simulink library "atmosphere_lib"  (R2018b)
settings: Solver=VariableStepAuto  StartTime=0.0  StopTime=10.0  RelTol=1e-3
values from neighbouring files (symbols this model uses):
  wg = interp1(y',wg_big',Y)'    [vonKarman2D.m]
  x = 0:Delta_x:x_max    [vonKarman1D.m]    (also in vonKarman2D.m)
undefined symbols (not defined in the file or in its folder): DiscIntNeverNeededParam
libraries: simulink x3, linear_systems_lib x3
settings Model: Creator=Ybeyer  LastModifiedBy=yannic
settings DebuggingCC: LibraryContextMissingDiagnostic=none
settings SFSimCC: SimUseLocalCustomCode=off
settings RTWCC: RTWUseLocalCustomCode=off
settings CodeAppCC: StateflowObjectComments=on

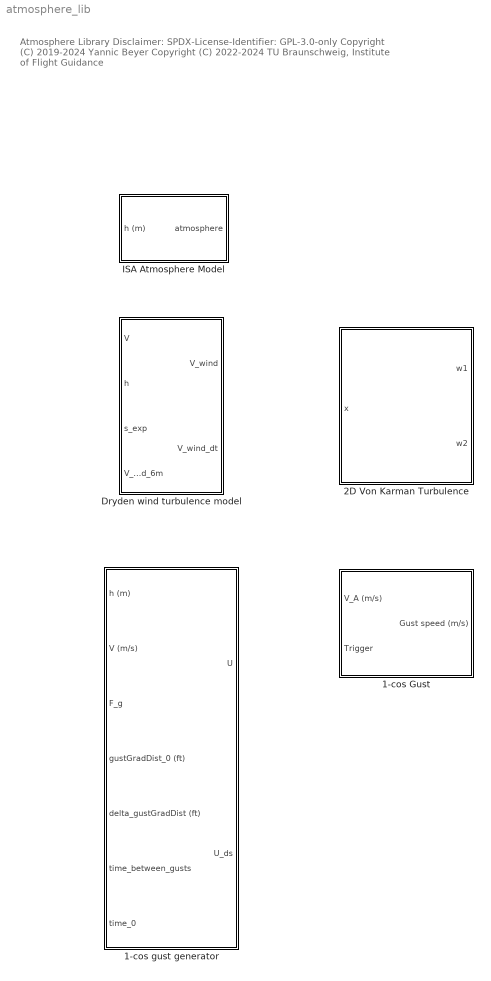
== system atmosphere_lib ==
  note: Atmosphere Library
      |
      | Disclaimer:
      | SPDX-License-Identifier: GPL-3.0-only
      |
      | Copyright (C) 2019-2024 Yannic Beyer
      | Copyright (C) 2022-2024 TU Braunschweig, Institute of Flight Guidance
  1-cos Gust : Subsystem  mask{gust_magnitude=3, gust_length=20}
      mask prompts: gust_magnitude "Gust magnitude, in m/s"; gust_length "Gust length, in m"
      mask DialogControl DescGroupVar Prompt: 1-cos gust
      mask DialogControl DescTextVar Prompt: This block creates 1-cos gust speeds.
  1-cos gust generator : Subsystem
      mask DialogControl DescGroupVar Prompt: 1-cos gust generator
      mask DialogControl DescTextVar Prompt: With this block you can generate a time series of 1-cos gusts. You can use the inputs to specify parameters like the initial gust gradient distance and how you want to increment the gust gradient distance for the next gust. Moreover, you can specify the time between the gusts.
      mask DialogControl ParameterGroupVar Prompt: Inputs
      mask DialogControl Control2 Prompt: h - altitude (m)
      mask DialogControl Control3 Prompt: V - airspeed of the aircraft (m/s)
      mask DialogControl Control4 Prompt: F_g - flight profile alleviation factor
      mask DialogControl Control5 Prompt: gustGradDist_0 - initial gust gradient distance (m)
      mask DialogControl Control6 Prompt: delta_gustGradDist - difference of the gust gradient distance for the next gust (m)
      mask DialogControl Control7 Prompt: time_between gusts - the time between gusts where there will be no wind (s)
      mask DialogControl Control8 Prompt: time_0 - time when the first gust starts
  2D Von Karman Turbulence : Subsystem  mask{x_max=10000, y_max=2*762, Delta_x=1, Delta_y=1, sigma=6.5, L=762, Y={[-2,-1,0,1,2],[-10,-5,0,5,10]}, is_symmetric=on, seed=2}
      mask prompts: x_max "Longitudinal length (m) - should be higher than scale length"; y_max "Lateral width (m) - should be higher than scale length"; Delta_x "Longitudinal position resolution (m)"; Delta_y "Lateral position resolution (m)"; sigma "Turbulence velocity variance (m/s), see turbulenceIntensityRMS"; L "Scale length at medium/high altitudes (m)"; Y "Lateral positions of interest (m)"; is_symmetric "Should the wind field be symmetric in lateral direction?"; seed "Noise seed"
      mask init:
      | y = [];
      | len = [];
      | for i = 1:length(Y)
      |     y(end+1:end+length(Y{i})) = Y{i};
      |     len(end+1) = length(Y{i});
      | end
      | [wg,wg_big,x] = vonKarman2D( x_max, y_max, Delta_x, Delta_y, y, sigma, L, seed, is_symmetric );
      | assignin('base','wind2D',wg);
      | assignin('base','wind2D_big',wg_big);
      | vonKarman2DInitBlock(gcb,len);
      mask DialogControl DescGroupVar Prompt: 2D von Kármán turbulence wind field
      mask DialogControl DescTextVar Prompt: For the 2D turbulence field no only computation via a white noise generator and a filter could be found. Instead, the wind field is computed during initialization with a 2D fourier transform according to literature.
      mask DialogControl Control2 Prompt: The whole wind field is saved to the base workspace as "wind2D_big". The wind field for the lateral positions of interest is saved as "wind2D".
  Dryden wind turbulence model : Subsystem  mask{noise_sample_time=0.01, noise_seed=[23341,23342,23343]}
      mask prompts: noise_sample_time "band-limited white noise sample time"; noise_seed "band-limited white noise seed"
      mask DialogControl DescTextVar Prompt: Inputs:
      mask DialogControl Control2 Prompt: V   - airspeed, m/s
      mask DialogControl Control3 Prompt: h   - altitude, m
      mask DialogControl Control4 Prompt: s_exp   - severity exponent (-1...6)
      mask DialogControl Control5 Prompt: V_wind   - wind velocity 6m above ground
  ISA Atmosphere Model : Subsystem
      mask init:
      | % init atmosphere struct
      | atmosphere = isAtmosphere(0);
      | % create bus object in base workspace
      | struct2bus(atmosphere);
      mask DialogControl DescGroupVar Prompt: International Standard Atmosphere Model
      mask DialogControl DescTextVar Prompt: The output is a bus (bus object is created in base workspace) and all quantities are in SI units.

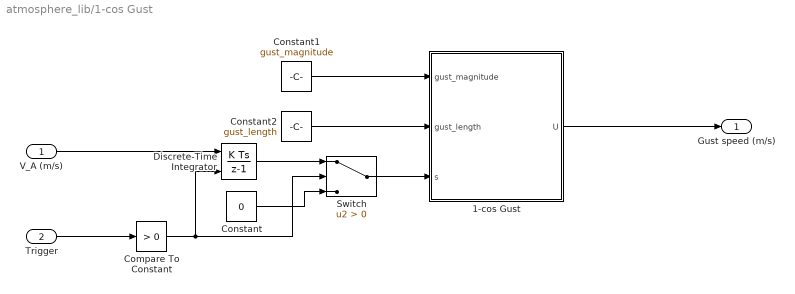
== system atmosphere_lib/1-cos Gust ==
  V_A (m/s) : Inport
  Trigger : Inport  Port=2
  1-cos Gust : MATLAB Function  TreatAsAtomicUnit=on
  Compare To Constant : simulink/Logic and Bit Operations/Compare To Constant  relop=>  const=0  OutDataTypeStr=boolean
  Constant : Constant  Value=0
  Constant1 : Constant  Value=gust_magnitude
  Constant2 : Constant  Value=gust_length
  Discrete-Time Integrator : DiscreteIntegrator  ExternalReset=rising  SampleTime=-1  ICPrevOutput=DiscIntNeverNeededParam  ICPrevScaledInput=DiscIntNeverNeededParam
  Switch : Switch  Criteria=u2 > Threshold
  Gust speed (m/s) : Outport
  wires:
  V_A (m/s)/1 -> Discrete-Time Integrator/1
  Constant2/1 -> 1-cos Gust/2(gust_length)
  Discrete-Time Integrator/1 -> Switch/1
  Trigger/1 -> Compare To Constant/1
  Compare To Constant/1 -> Switch/2, Discrete-Time Integrator/2
  Switch/1 -> 1-cos Gust/3(s)
  Constant/1 -> Switch/3
  1-cos Gust/1(U) -> Gust speed (m/s)/1
  Constant1/1 -> 1-cos Gust/1(gust_magnitude)

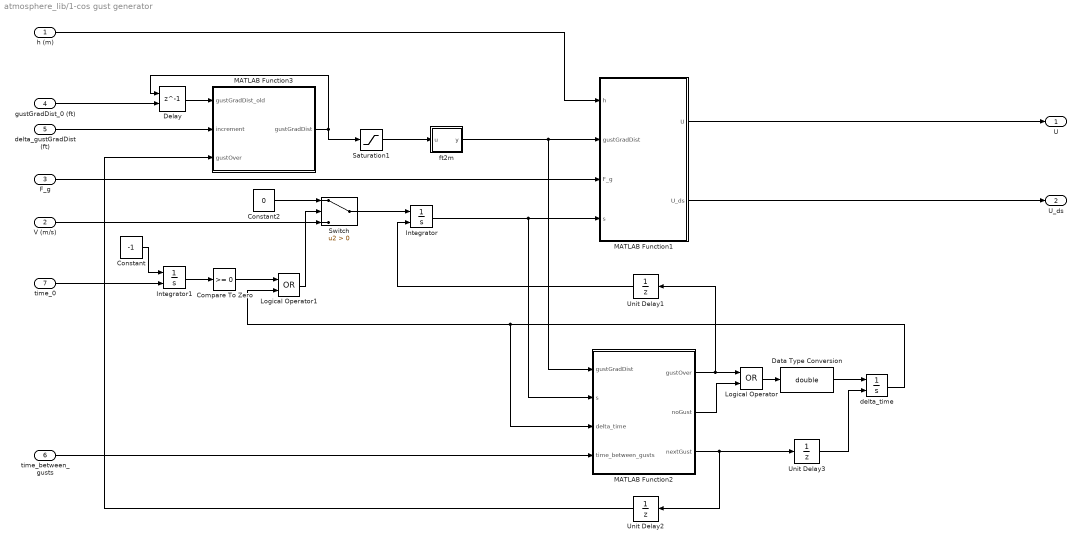
== system atmosphere_lib/1-cos gust generator ==
  h (m) : Inport
  V (m/s) : Inport  Port=2
  F_g : Inport  Port=3
  gustGradDist_0 (ft) : Inport  Port=4
  delta_gustGradDist (ft) : Inport  Port=5
  time_between_gusts : Inport  Port=6
  time_0 : Inport  Port=7
  Compare To Zero : simulink/Logic and Bit Operations/Compare To Zero  relop=>=  OutDataTypeStr=boolean
  Constant : Constant  Value=-1
  Constant2 : Constant  Value=0
  Data Type Conversion : DataTypeConversion  OutDataTypeStr=double
  Delay : Delay  DelayLength=1  InitialConditionSource=Input port
      settings: InputPortMap=u0,p4
  Integrator : Integrator  ExternalReset=rising
  Integrator1 : Integrator  InitialConditionSource=external
  Logical Operator : Logic  Operator=OR  AllPortsSameDT=off  OutDataTypeStr=boolean
  Logical Operator1 : Logic  Operator=OR  AllPortsSameDT=off  OutDataTypeStr=boolean
  MATLAB Function1 : MATLAB Function  TreatAsAtomicUnit=on
  MATLAB Function2 : MATLAB Function  TreatAsAtomicUnit=on
  MATLAB Function3 : MATLAB Function  TreatAsAtomicUnit=on
  Saturation1 : Saturate  UpperLimit=349.9  LowerLimit=30.1
  Switch : Switch  Criteria=u2 > Threshold
  Unit Delay1 : UnitDelay  SampleTime=-1
  Unit Delay2 : UnitDelay  SampleTime=-1
  Unit Delay3 : UnitDelay  SampleTime=-1
  delta_time : Integrator  ExternalReset=rising
  ft2m : MATLAB Function  TreatAsAtomicUnit=on
  U : Outport
  U_ds : Outport  Port=2
  wires:
  delta_gustGradDist (ft)/1 -> MATLAB Function3/2(increment)
  MATLAB Function1/1(U) -> U/1
  Saturation1/1 -> ft2m/1(u)
  h (m)/1 -> MATLAB Function1/1(h)
  F_g/1 -> MATLAB Function1/3(F_g)
  MATLAB Function1/2(U_ds) -> U_ds/1
  ft2m/1(y) -> MATLAB Function1/2(gustGradDist), MATLAB Function2/1(gustGradDist)
  MATLAB Function3/1(gustGradDist) -> Saturation1/1, Delay/1
  Integrator/1 -> MATLAB Function1/4(s), MATLAB Function2/2(s)
  V (m/s)/1 -> Switch/3
  Switch/1 -> Integrator/1
  Constant2/1 -> Switch/1
  time_between_gusts/1 -> MATLAB Function2/4(time_between_gusts)
  MATLAB Function2/2(noGust) -> Logical Operator/2
  Logical Operator/1 -> Data Type Conversion/1
  MATLAB Function2/1(gustOver) -> Logical Operator/1, Unit Delay1/1
  MATLAB Function2/3(nextGust) -> Unit Delay3/1, Unit Delay2/1
  Data Type Conversion/1 -> delta_time/1
  Unit Delay1/1 -> Integrator/2
  Unit Delay2/1 -> MATLAB Function3/3(gustOver)
  delta_time/1 -> Logical Operator1/2, MATLAB Function2/3(delta_time)
  Unit Delay3/1 -> delta_time/2
  Delay/1 -> MATLAB Function3/1(gustGradDist_old)
  gustGradDist_0 (ft)/1 -> Delay/2
  Constant/1 -> Integrator1/1
  time_0/1 -> Integrator1/2
  Logical Operator1/1 -> Switch/2
  Integrator1/1 -> Compare To Zero/1
  Compare To Zero/1 -> Logical Operator1/1

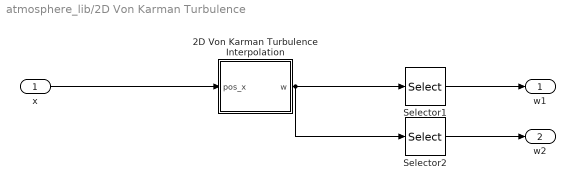
== system atmosphere_lib/2D Von Karman Turbulence ==
  x : Inport
  2D Von Karman Turbulence Interpolation : MATLAB Function  TreatAsAtomicUnit=on
  Selector1 : Selector  InputPortWidth=10  IndexOptions=Index vector (dialog)  Indices=1:5  OutputSizes=1
  Selector2 : Selector  InputPortWidth=10  IndexOptions=Index vector (dialog)  Indices=6:10  OutputSizes=1
  w1 : Outport
  w2 : Outport  Port=2
  wires:
  2D Von Karman Turbulence Interpolation/1(w) -> Selector1/1, Selector2/1
  x/1 -> 2D Von Karman Turbulence Interpolation/1(pos_x)
  Selector1/1 -> w1/1
  Selector2/1 -> w2/1

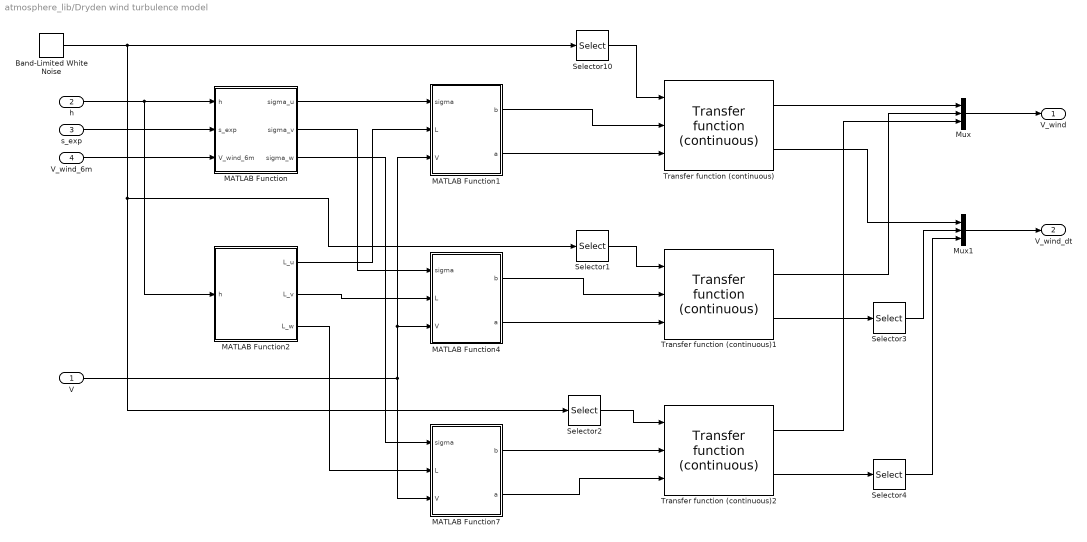
== system atmosphere_lib/Dryden wind turbulence model ==
  V : Inport
  h : Inport  Port=2
  s_exp : Inport  Port=3
  V_wind_6m : Inport  Port=4
  Band-Limited White Noise : simulink/Sources/Band-Limited White Noise  Cov=[1,1,1]*pi  Ts=noise_sample_time  seed=noise_seed
  MATLAB Function : MATLAB Function  TreatAsAtomicUnit=on
  MATLAB Function1 : MATLAB Function  TreatAsAtomicUnit=on
  MATLAB Function2 : MATLAB Function  TreatAsAtomicUnit=on
  MATLAB Function4 : MATLAB Function  TreatAsAtomicUnit=on
  MATLAB Function7 : MATLAB Function  TreatAsAtomicUnit=on
  Mux : Mux  Inputs=3
  Mux1 : Mux  Inputs=3
  Selector1 : Selector  InputPortWidth=3  IndexOptions=Index vector (dialog)  Indices=2  OutputSizes=1
  Selector10 : Selector  InputPortWidth=3  IndexOptions=Index vector (dialog)  Indices=1  OutputSizes=1
  Selector2 : Selector  InputPortWidth=3  IndexOptions=Index vector (dialog)  Indices=3  OutputSizes=1
  Selector3 : Selector  InputPortWidth=2  IndexOptions=Index vector (dialog)  Indices=2  OutputSizes=1
  Selector4 : Selector  InputPortWidth=2  IndexOptions=Index vector (dialog)  Indices=2  OutputSizes=1
  Transfer function (continuous) : linear_systems_lib/Transfer function (continuous)
      settings: SourceProductName=LADAC
  Transfer function (continuous)1 : linear_systems_lib/Transfer function (continuous)
      settings: SourceProductName=LADAC
  Transfer function (continuous)2 : linear_systems_lib/Transfer function (continuous)
      settings: SourceProductName=LADAC
  V_wind : Outport
  V_wind_dt : Outport  Port=2
  wires:
  MATLAB Function2/1(L_u) -> MATLAB Function1/2(L)
  MATLAB Function/1(sigma_u) -> MATLAB Function1/1(sigma)
  Mux/1 -> V_wind/1
  MATLAB Function/2(sigma_v) -> MATLAB Function4/1(sigma)
  MATLAB Function1/2(a) -> Transfer function (continuous)/3
  MATLAB Function4/1(b) -> Transfer function (continuous)1/2
  Selector3/1 -> Mux1/2
  MATLAB Function2/3(L_w) -> MATLAB Function7/2(L)
  Selector4/1 -> Mux1/3
  MATLAB Function1/1(b) -> Transfer function (continuous)/2
  MATLAB Function7/1(b) -> Transfer function (continuous)2/2
  Mux1/1 -> V_wind_dt/1
  MATLAB Function7/2(a) -> Transfer function (continuous)2/3
  h/1 -> MATLAB Function2/1(h), MATLAB Function/1(h)
  Selector1/1 -> Transfer function (continuous)1/1
  s_exp/1 -> MATLAB Function/2(s_exp)
  Band-Limited White Noise/1 -> Selector2/1, Selector1/1, Selector10/1
  V/1 -> MATLAB Function1/3(V), MATLAB Function4/3(V), MATLAB Function7/3(V)
  Selector2/1 -> Transfer function (continuous)2/1
  V_wind_6m/1 -> MATLAB Function/3(V_wind_6m)
  MATLAB Function4/2(a) -> Transfer function (continuous)1/3
  MATLAB Function2/2(L_v) -> MATLAB Function4/2(L)
  MATLAB Function/3(sigma_w) -> MATLAB Function7/1(sigma)
  Transfer function (continuous)1/2 -> Selector3/1
  Transfer function (continuous)/1 -> Mux/1
  Selector10/1 -> Transfer function (continuous)/1
  Transfer function (continuous)/2 -> Mux1/1
  Transfer function (continuous)1/1 -> Mux/2
  Transfer function (continuous)2/1 -> Mux/3
  Transfer function (continuous)2/2 -> Selector4/1

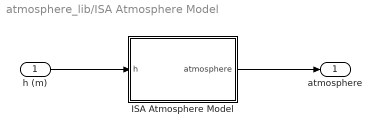
== system atmosphere_lib/ISA Atmosphere Model ==
  h (m) : Inport
  ISA Atmosphere Model : MATLAB Function  TreatAsAtomicUnit=on
  atmosphere : Outport
  wires:
  h (m)/1 -> ISA Atmosphere Model/1(h)
  ISA Atmosphere Model/1(atmosphere) -> atmosphere/1

== matlab function atmosphere_lib/Dryden wind turbulence model/MATLAB Function1 ==
  data: sigma input; b output; L input; V input; a output
function [b,a] = drydenTf( sigma, L, V ) %#codegen
[b,a] = drydenTf( sigma, L, V, 'u' );
end

== matlab function atmosphere_lib/ISA Atmosphere Model/ISA Atmosphere Model ==
  data: h input; atmosphere output Bus: atmosphere_bus
function atmosphere = isAtmosphere( h ) %#codegen
atmosphere = isAtmosphere( h );
end

== matlab function atmosphere_lib/Dryden wind turbulence model/MATLAB Function ==
  data: h input; sigma_u output; s_exp input; V_wind_6m input; sigma_v output; sigma_w output
function [ sigma_u, sigma_v, sigma_w ] = fcn( h, s_exp, V_wind_6m ) %#codegen
[ sigma_u, sigma_v, sigma_w ] = turbulenceIntensityRMS( h, s_exp, V_wind_6m );
end

== matlab function atmosphere_lib/Dryden wind turbulence model/MATLAB Function2 ==
  data: h input; L_u output; L_v output; L_w output
function [ L_u, L_v, L_w ] = fcn( h ) %#codegen
[ L_u, L_v, L_w ] = turbulenceScaleLength( h );
end

== matlab function atmosphere_lib/Dryden wind turbulence model/MATLAB Function4 ==
  data: sigma input; b output; L input; V input; a output
function [b,a] = drydenTf( sigma, L, V ) %#codegen
[b,a] = drydenTf( sigma, L, V, 'v' );
end

== matlab function atmosphere_lib/1-cos gust generator/MATLAB Function1 ==
  data: h input; U output; gustGradDist input; F_g input; s input; U_ds output
function [U,U_ds] = fcn(h,gustGradDist,F_g,s)

% define 1-cos gust
U_ref           = oneMinusCosGustUref( h );
U_ds            = oneMinusCosGustUds( U_ref, gustGradDist, F_g );
U               = U_ds/2 * ( 1 - cos( pi*s/gustGradDist ) );

end

== matlab function atmosphere_lib/1-cos gust generator/MATLAB Function2 ==
  data: gustGradDist input; gustOver output; s input; delta_time input; time_between_gusts input; noGust output; nextGust output
function [ gustOver, noGust, nextGust ] = fcn(gustGradDist, s, delta_time,time_between_gusts) %#codegen

if s >= 2*gustGradDist
    gustOver = 1;
else
    gustOver = 0;
end

if  delta_time > 0 && delta_time < time_between_gusts
    noGust = 1;
else
    noGust = 0;
end

if delta_time >= time_between_gusts
    nextGust = 1;
else
    nextGust = 0;
end

end

== matlab function atmosphere_lib/Dryden wind turbulence model/MATLAB Function7 ==
  data: sigma input; b output; L input; V input; a output
function [b,a] = drydenTf( sigma, L, V ) %#codegen
[b,a] = drydenTf( sigma, L, V, 'w' );
end

== matlab function atmosphere_lib/1-cos gust generator/MATLAB Function3 ==
  data: gustGradDist_old input; increment input; gustGradDist output; gustOver input
function gustGradDist = fcn( gustGradDist_old, increment, gustOver ) %#codegen

if gustOver
    gustGradDist = gustGradDist_old + increment;
else
    gustGradDist = gustGradDist_old;
end

== matlab function atmosphere_lib/1-cos gust generator/ft2m ==
  data: u input; y output
function y = fcn(u)
y = ft2m(u);

== matlab function atmosphere_lib/2D Von Karman Turbulence/2D Von Karman Turbulence Interpolation ==
  data: pos_x input; w output; wg parameter; x parameter
function w = fcn(pos_x,wg, x)
w = zeros(size(wg,2),1);
if pos_x<x(end)
    w(:) = interp1(x(:),wg,pos_x);
    w(isnan(w))=0;
end
end

== matlab function atmosphere_lib/1-cos Gust/1-cos Gust ==
  data: gust_magnitude input; U output; gust_length input; s input
function U = fcn(gust_magnitude,gust_length,s)
U = zeros(1,class(s));
cos_arg = 2*pi*s/gust_length;
if cos_arg > 0 && cos_arg <= 2*pi
    U(:) = gust_magnitude/2 * ( 1 - cos( cos_arg ) );
end
end
